simulink model "mod_03"  (R2025a)
settings: Solver=ode45  StartTime=0.0  StopTime=40  MaxStep=1e-2  RelTol=1e-3
values from neighbouring files (symbols this model uses):
  B = 1000    [codigo_mod03.m]
  K = 50000    [codigo_mod03.m]
  M = 100    [codigo_mod03.m]
settings Model: Creator=fabri  LastModifiedBy=fabri

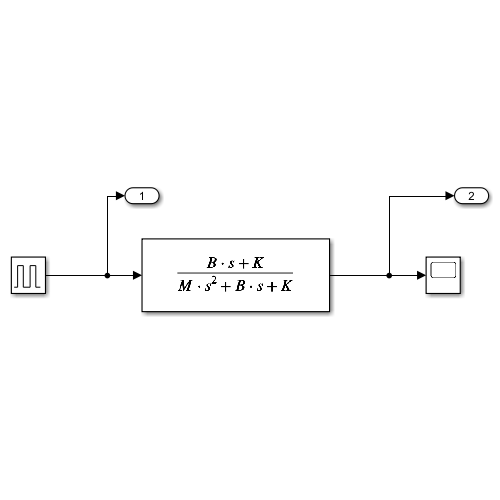
[thumbnail: Simulink's stored preview of the top-level diagram]
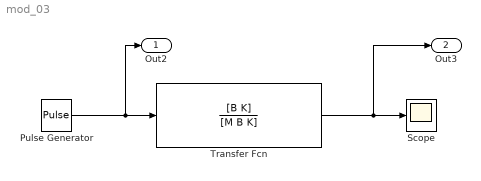
== system mod_03 ==
  Pulse Generator : DiscretePulseGenerator  PulseType=Time based  Amplitude=0.8  Period=10  PulseWidth=50
  Scope : Scope
      settings: ActiveDisplayYMinimum=-1.7458003967535334  ActiveDisplayYMaximum=2.0268826752874971
  Transfer Fcn : TransferFcn  Numerator=[B K]  Denominator=[M B K]
  Out2 : Outport
  Out3 : Outport  Port=2
  wires:
  Pulse Generator/1 -> Out2/1, Transfer Fcn/1
  Transfer Fcn/1 -> Out3/1, Scope/1
